simulink model "sf_cpp"  (R2025b)
settings: Solver=FixedStepDiscrete  StartTime=0.0  StopTime=100  FixedStep=1  RelTol=1e-3  EnableMultiTasking=on
settings Model: FPTRunName=Active  ExtModeAutoUpdateStatusClock=off  Creator=The MathWorks, Inc.  LastModifiedBy=The MathWorks, Inc.
settings SolverCC: AlgebraicLoopSolver=TrustRegion  MaxZcPerStep=1.0
settings DataIOCC: LimitDataPoints=on  SaveFormat=Array  SaveOutput=off  SaveTime=off  ReturnWorkspaceOutputs=off  SignalLoggingName=sigsOut
settings OptimizationCC: DefaultParameterBehavior=Inlined  InlineInvariantSignals=on  ReuseModelBlockBuffer=off  ExpressionDepthLimit=2147483647.0  StateBitsets=on  DataBitsets=on  ZeroExternalMemoryAtStartup=off  ZeroInternalMemoryAtStartup=off  InitFltsAndDblsToZero=on  LifeSpan=inf  BufferReusableBoundary=off
settings DebuggingCC: SaveWithParameterizedLinksMsg=none  UnderspecifiedInitializationDetection=Classic  MergeDetectMultiDrivingBlocksExec=none  CheckExecutionContextPreStartOutputMsg=on  SignalResolutionControl=TryResolveAllWithWarning  MultiTaskDSMMsg=warning  MultiTaskCondExecSysMsg=none  FcnCallInpInsideContextMsg=warning  UnconnectedInputMsg=warning  UnconnectedOutputMsg=warning  UnconnectedLineMsg=warning  StateNameClashWarn=warning  SFUnexpectedBacktrackingDiag=warning  SFNoUnconditionalDefaultTransitionDiag=warning  SFExecutionAtInitializationDiag=none  ArithmeticOperatorsInVariantConditions=warning
settings HardwareCC: ProdBitPerPointer=32.0  ProdBitPerSizeT=32.0  ProdBitPerPtrDiffT=32.0  ProdLargestAtomicFloat=None  ProdIntDivRoundTo=Undefined  ProdEndianess=Unspecified  ProdWordSize=32.0  ProdHWDeviceType=32-bit Generic  TargetHWDeviceType=32-bit Generic
settings ModelReferenceCC: EnableRefExpFcnMdlSchedulingChecks=on  PropagateSignalLabelsOutOfModel=off
settings SFSimCC: SimCustomInitializer=adderVar = createAdder();  SimCustomTerminator=deleteAdder(adderVar);  SimUseLocalCustomCode=off  CustomCodeUndefinedFunction=UseInterfaceOnly  SimTargetLang=C++  SimDLTargetLibrary=mkl-dnn
settings SFSimCC: SimCustomHeaderCode=|
  | #include "adder_cpp.h"
  | #include "adder_wrapper.h"
settings SFSimCC: SimUserSources=|
  | adder_cpp.cpp
  | adder_wrapper.cpp
settings RTWCC: GenerateReport=on  RTWVerbose=off  RTWUseLocalCustomCode=off  RTWUseSimCustomCode=on  CustomInitializer=adderVar = createAdder();  CustomTerminator=deleteAdder(adderVar);  LaunchReport=on  TargetLang=C++  GPUComputeCapability=3.5  DLArmComputeVersion=19.05
settings RTWCC: CustomHeaderCode=|
  | #include "adder_cpp.h"
  | #include "adder_wrapper.h"
settings RTWCC: CustomSource=|
  | adder_cpp.cpp
  | adder_wrapper.cpp
settings CodeAppCC: ForceParamTrailComments=on  StateflowObjectComments=on
settings GRTTargetCC: TargetFcnLib=ansi_tfl_tmw.mat  TargetLangStandard=C++11 (ISO)  MatFileLogging=off  CodeInterfacePackaging=C++ class  SubcomponentCodeInterfacePackaging=C++ class
settings ConfigComp: CovScope=ReferencedModels  CovMetricSettings=dcmtr  CovSaveCumulativeToWorkspaceVar=on  CovSaveSingleToWorkspaceVar=on  CovExternalEMLEnable=off  CovSFcnEnable=off

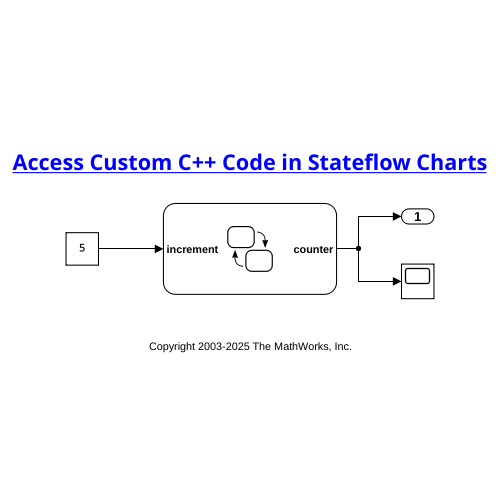
[thumbnail: Simulink's stored preview of the top-level diagram]
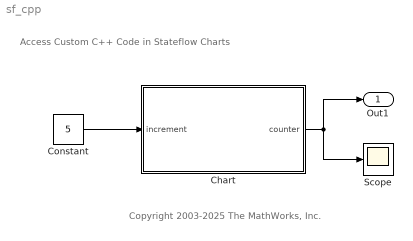
== system sf_cpp ==
  note: Copyright 2003-2025 The MathWorks, Inc.
  note: Access Custom C++ Code in Stateflow Charts
  Chart : Stateflow chart  TreatAsAtomicUnit=on
  Constant : Constant  Value=5  OutDataTypeStr=int32
  Scope : Scope
      settings: ActiveDisplayYMaximum=110
  Out1 : Outport  VectorParamsAs1DForOutWhenUnconnected=off
  wires:
  Constant/1 -> Chart/1(increment)
  Chart/1(counter) -> Scope/1, Out1/1

== stateflow chart sf_cpp/Chart ==
  state Increase
    during: counter = adderOutput(adderVar,increment);
  state Decrease
    during: counter = adderOutput(adderVar,-increment);
  (default) -> Increase : {counter = 0;}
  Decrease -> Increase : [counter <= 100]
  Increase -> Decrease : [counter > 100]
  data: counter output double; increment input
